simulink model "modele_qpsk_codee"  (R2024b)
settings: Solver=FixedStepDiscrete  StartTime=0.0  StopTime=(Nsim-1)*Tb  FixedStep=Tpas  RelTol=1e-3
undefined symbols (not defined in the file or in its folder): dAlign, graine, mappingGray, N0, phaseC, Tb, Tc, Tsym
settings Model: Creator=youka  LastModifiedBy=youka

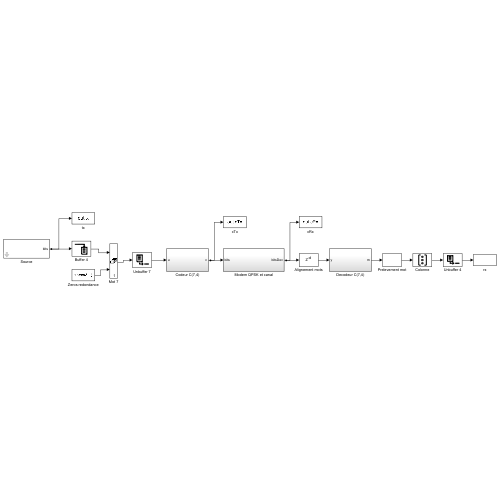
[thumbnail: Simulink's stored preview of the top-level diagram]
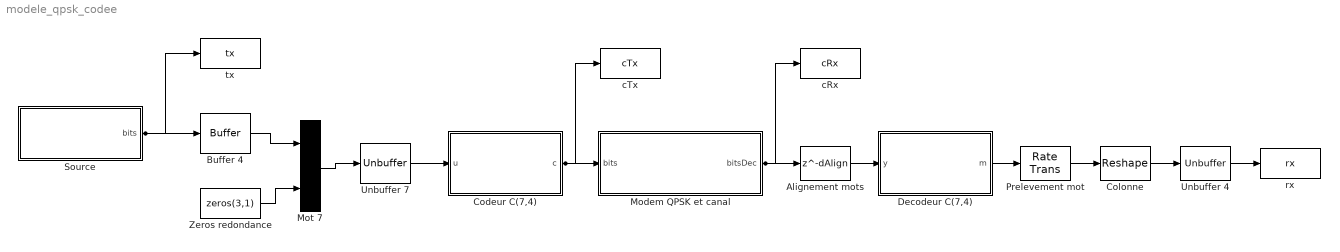
== system modele_qpsk_codee ==
  Alignement mots : Delay  DelayLength=dAlign
  Buffer 4 : Buffer  N=4
  Codeur C(7,4) : Subsystem
  Colonne : Reshape  OutputDimensionality=Column vector (2-D)
  Decodeur C(7,4) : Subsystem
  Modem QPSK et canal : Subsystem
  Mot 7 : Concatenate  Mode=Multidimensional array
  Prelevement mot : RateTransition  OutPortSampleTime=4*Tb
  Source : Subsystem  mask(Source binaire){p_m=0.5, Tb_m=Tb, graine_m=graine}
      mask prompts: p_m "Probabilité d'émettre un 1"; Tb_m "Durée d'un bit Tb (s)"; graine_m "Graine (Seed)"
      mask help: Source binaire sans mémoire : P(1) = p, un bit toutes les Tb secondes.
  Unbuffer 4 : Unbuffer
  Unbuffer 7 : Unbuffer
  Zeros redondance : Constant  Value=zeros(3,1)  SampleTime=4*Tb
  cRx : ToWorkspace  VariableName=cRx  SampleTime=-1
  cTx : ToWorkspace  VariableName=cTx  SampleTime=-1
  rx : ToWorkspace  VariableName=rx  SampleTime=-1
  tx : ToWorkspace  VariableName=tx  SampleTime=-1
  wires:
  Source/1(bits) -> tx/1, Buffer 4/1
  Buffer 4/1 -> Mot 7/1
  Zeros redondance/1 -> Mot 7/2
  Mot 7/1 -> Unbuffer 7/1
  Unbuffer 7/1 -> Codeur C(7,4)/1(u)
  Codeur C(7,4)/1(c) -> cTx/1, Modem QPSK et canal/1(bits)
  Modem QPSK et canal/1(bitsDec) -> cRx/1, Alignement mots/1
  Alignement mots/1 -> Decodeur C(7,4)/1(y)
  Decodeur C(7,4)/1(m) -> Prelevement mot/1
  Prelevement mot/1 -> Colonne/1
  Colonne/1 -> Unbuffer 4/1
  Unbuffer 4/1 -> rx/1

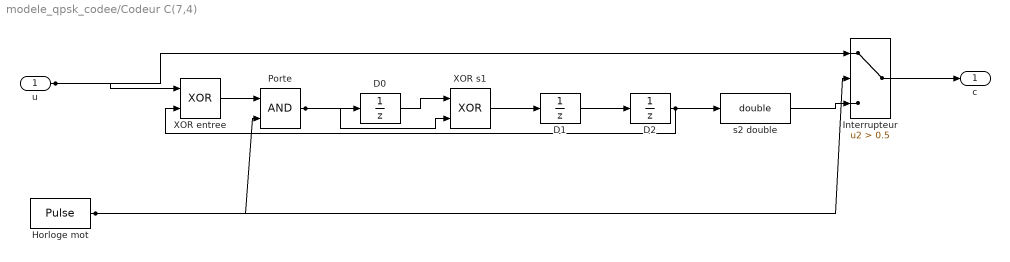
== system modele_qpsk_codee/Codeur C(7,4) ==
  u : Inport
  D0 : UnitDelay  SampleTime=Tc  HasFrameUpgradeWarning=on
  D1 : UnitDelay  SampleTime=Tc  HasFrameUpgradeWarning=on
  D2 : UnitDelay  SampleTime=Tc  HasFrameUpgradeWarning=on
  Horloge mot : DiscretePulseGenerator  Period=7  PulseWidth=4  PhaseDelay=phaseC  SampleTime=Tc
  Interrupteur : Switch  Criteria=u2 > Threshold  Threshold=0.5  SaturateOnIntegerOverflow=off  InputSameDT=off
  Porte : Logic  AllPortsSameDT=off  OutDataTypeStr=boolean
  XOR entree : Logic  Operator=XOR  AllPortsSameDT=off  OutDataTypeStr=boolean
  XOR s1 : Logic  Operator=XOR  AllPortsSameDT=off  OutDataTypeStr=boolean
  s2 double : DataTypeConversion  OutDataTypeStr=double  SaturateOnIntegerOverflow=off  RndMeth=Floor
  c : Outport
  wires:
  u/1 -> XOR entree/1, Interrupteur/1
  D2/1 -> XOR entree/2, s2 double/1
  XOR entree/1 -> Porte/1
  Horloge mot/1 -> Porte/2, Interrupteur/2
  Porte/1 -> D0/1, XOR s1/2
  D0/1 -> XOR s1/1
  XOR s1/1 -> D1/1
  D1/1 -> D2/1
  s2 double/1 -> Interrupteur/3
  Interrupteur/1 -> c/1

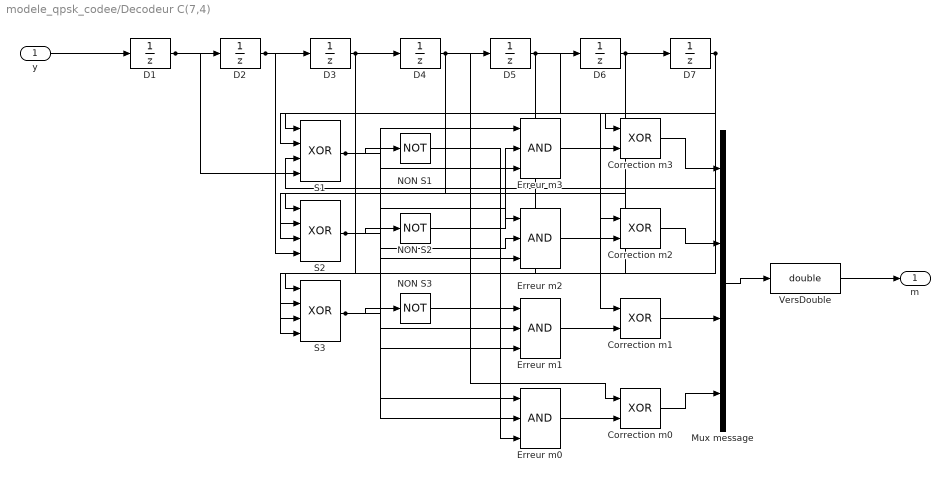
== system modele_qpsk_codee/Decodeur C(7,4) ==
  y : Inport
  Correction m{0..3} (4 alike) : Logic  Operator=XOR  AllPortsSameDT=off  OutDataTypeStr=boolean
  D{1..7} (7 alike) : UnitDelay  SampleTime=Tc  HasFrameUpgradeWarning=on
  Erreur m{0..3} (4 alike) : Logic  Inputs=3  AllPortsSameDT=off  OutDataTypeStr=boolean
  Mux message : Mux
  NON S1 : Logic  Operator=NOT  AllPortsSameDT=off  OutDataTypeStr=boolean
  NON S2 : Logic  Operator=NOT  AllPortsSameDT=off  OutDataTypeStr=boolean
  NON S3 : Logic  Operator=NOT  AllPortsSameDT=off  OutDataTypeStr=boolean
  S1 : Logic  Operator=XOR  Inputs=4  AllPortsSameDT=off  OutDataTypeStr=boolean
  S2 : Logic  Operator=XOR  Inputs=4  AllPortsSameDT=off  OutDataTypeStr=boolean
  S3 : Logic  Operator=XOR  Inputs=4  AllPortsSameDT=off  OutDataTypeStr=boolean
  VersDouble : DataTypeConversion  OutDataTypeStr=double  SaturateOnIntegerOverflow=off  RndMeth=Floor
  m : Outport
  wires:
  y/1 -> D1/1
  D1/1 -> D2/1, S1/4
  D2/1 -> D3/1, S2/4
  D3/1 -> D4/1, S3/4
  D4/1 -> D5/1, S1/1, S2/1, Correction m0/1
  D5/1 -> D6/1, S2/2, S3/1, Correction m1/1
  D6/1 -> D7/1, S1/2, S2/3, S3/2, Correction m2/1
  D7/1 -> S1/3, S3/3, Correction m3/1
  S1/1 -> NON S1/1, Erreur m3/1, Erreur m2/1, Erreur m0/1
  S2/1 -> NON S2/1, Erreur m2/2, Erreur m1/2, Erreur m0/2
  S3/1 -> NON S3/1, Erreur m3/3, Erreur m2/3, Erreur m1/3
  NON S2/1 -> Erreur m3/2
  Erreur m3/1 -> Correction m3/2
  Erreur m2/1 -> Correction m2/2
  NON S1/1 -> Erreur m1/1
  Erreur m1/1 -> Correction m1/2
  NON S3/1 -> Erreur m0/3
  Erreur m0/1 -> Correction m0/2
  Correction m3/1 -> Mux message/1
  Correction m2/1 -> Mux message/2
  Correction m1/1 -> Mux message/3
  Correction m0/1 -> Mux message/4
  Mux message/1 -> VersDouble/1
  VersDouble/1 -> m/1

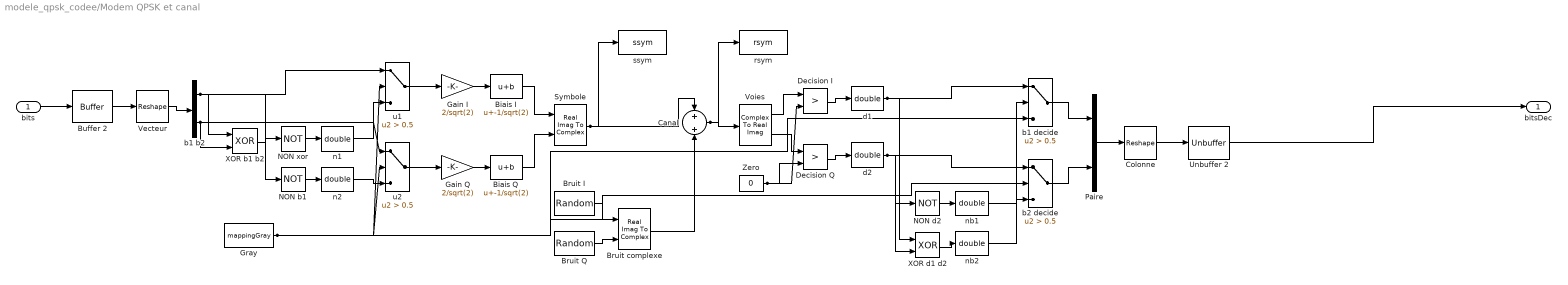
== system modele_qpsk_codee/Modem QPSK et canal ==
  bits : Inport
  Biais I : Bias  Bias=-1/sqrt(2)  SaturateOnIntegerOverflow=off
  Biais Q : Bias  Bias=-1/sqrt(2)  SaturateOnIntegerOverflow=off
  Bruit I : RandomNumber  Variance=N0/2  Seed=graine+1  SampleTime=Tsym
  Bruit Q : RandomNumber  Variance=N0/2  Seed=graine+2  SampleTime=Tsym
  Bruit complexe : RealImagToComplex
  Buffer 2 : Buffer  N=2
  Canal : Sum
  Colonne : Reshape  OutputDimensionality=Column vector (2-D)
  Decision I : RelationalOperator  Operator=>  OutDataTypeStr=boolean  RndMeth=Simplest  InputSameDT=off
  Decision Q : RelationalOperator  Operator=>  OutDataTypeStr=boolean  RndMeth=Simplest  InputSameDT=off
  Gain I : Gain  Gain=2/sqrt(2)
  Gain Q : Gain  Gain=2/sqrt(2)
  Gray : Constant  Value=mappingGray
  NON b1 : Logic  Operator=NOT  AllPortsSameDT=off  OutDataTypeStr=boolean
  NON d2 : Logic  Operator=NOT  AllPortsSameDT=off  OutDataTypeStr=boolean
  NON xor : Logic  Operator=NOT  AllPortsSameDT=off  OutDataTypeStr=boolean
  Paire : Mux  Inputs=2
  Symbole : RealImagToComplex
  Unbuffer 2 : Unbuffer
  Vecteur : Reshape
  Voies : ComplexToRealImag
  XOR b1 b2 : Logic  Operator=XOR  AllPortsSameDT=off  OutDataTypeStr=boolean
  XOR d1 d2 : Logic  Operator=XOR  AllPortsSameDT=off  OutDataTypeStr=boolean
  Zero : Constant  Value=0
  b1 b2 : Demux  Outputs=2
  b1 decide : Switch  Criteria=u2 > Threshold  Threshold=0.5  SaturateOnIntegerOverflow=off  InputSameDT=off
  b2 decide : Switch  Criteria=u2 > Threshold  Threshold=0.5  SaturateOnIntegerOverflow=off  InputSameDT=off
  d1 : DataTypeConversion  OutDataTypeStr=double  SaturateOnIntegerOverflow=off  RndMeth=Floor
  d2 : DataTypeConversion  OutDataTypeStr=double  SaturateOnIntegerOverflow=off  RndMeth=Floor
  n1 : DataTypeConversion  OutDataTypeStr=double  SaturateOnIntegerOverflow=off  RndMeth=Floor
  n2 : DataTypeConversion  OutDataTypeStr=double  SaturateOnIntegerOverflow=off  RndMeth=Floor
  nb1 : DataTypeConversion  OutDataTypeStr=double  SaturateOnIntegerOverflow=off  RndMeth=Floor
  nb2 : DataTypeConversion  OutDataTypeStr=double  SaturateOnIntegerOverflow=off  RndMeth=Floor
  rsym : ToWorkspace  VariableName=rsym  SampleTime=-1
  ssym : ToWorkspace  VariableName=ssym  SampleTime=-1
  u1 : Switch  Criteria=u2 > Threshold  Threshold=0.5  SaturateOnIntegerOverflow=off  InputSameDT=off
  u2 : Switch  Criteria=u2 > Threshold  Threshold=0.5  SaturateOnIntegerOverflow=off  InputSameDT=off
  bitsDec : Outport
  wires:
  bits/1 -> Buffer 2/1
  Buffer 2/1 -> Vecteur/1
  Vecteur/1 -> b1 b2/1
  b1 b2/1 -> XOR b1 b2/1, NON b1/1, u1/1
  b1 b2/2 -> XOR b1 b2/2, u2/1
  XOR b1 b2/1 -> NON xor/1
  NON xor/1 -> n1/1
  NON b1/1 -> n2/1
  Gray/1 -> u1/2, u2/2, b1 decide/2, b2 decide/2
  n1/1 -> u1/3
  n2/1 -> u2/3
  u1/1 -> Gain I/1
  Gain I/1 -> Biais I/1
  Biais I/1 -> Symbole/1
  u2/1 -> Gain Q/1
  Gain Q/1 -> Biais Q/1
  Biais Q/1 -> Symbole/2
  Bruit I/1 -> Bruit complexe/1
  Bruit Q/1 -> Bruit complexe/2
  Symbole/1 -> Canal/1, ssym/1
  Bruit complexe/1 -> Canal/2
  Canal/1 -> rsym/1, Voies/1
  Voies/1 -> Decision I/1
  Zero/1 -> Decision I/2, Decision Q/2
  Voies/2 -> Decision Q/1
  Decision I/1 -> d1/1
  Decision Q/1 -> d2/1
  d2/1 -> NON d2/1, XOR d1 d2/2, b2 decide/1
  NON d2/1 -> nb1/1
  d1/1 -> XOR d1 d2/1, b1 decide/1
  XOR d1 d2/1 -> nb2/1
  nb1/1 -> b1 decide/3
  nb2/1 -> b2 decide/3
  b1 decide/1 -> Paire/1
  b2 decide/1 -> Paire/2
  Paire/1 -> Colonne/1
  Colonne/1 -> Unbuffer 2/1
  Unbuffer 2/1 -> bitsDec/1

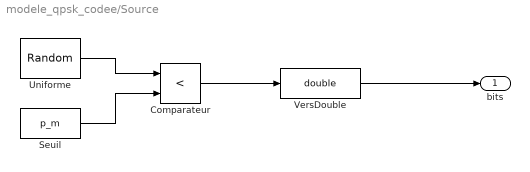
== system modele_qpsk_codee/Source ==
  Comparateur : RelationalOperator  Operator=<  OutDataTypeStr=boolean  RndMeth=Simplest  InputSameDT=off
  Seuil : Constant  Value=p_m  SampleTime=Tb_m
  Uniforme : UniformRandomNumber  Minimum=0  Seed=graine_m  SampleTime=Tb_m
  VersDouble : DataTypeConversion  OutDataTypeStr=double  SaturateOnIntegerOverflow=off  RndMeth=Floor
  bits : Outport
  wires:
  Uniforme/1 -> Comparateur/1
  Seuil/1 -> Comparateur/2
  Comparateur/1 -> VersDouble/1
  VersDouble/1 -> bits/1
